simulink model "beaver_agent_env"  (R2022a)
settings: Solver=VariableStepAuto  StartTime=0.0  StopTime=60  FixedStep=1/120  RelTol=1e-5
PreLoadFcn:
  | [aircraft, state] = astDehavillandBeaver();
  | thrustX = getCoefficient(aircraft,"CX","Propeller",Component="Propeller");
  | AileronCmd = 0.00202547955338193;
  | ElevatorCmd = -0.0109658218633661;
  | RudderCmd = -0.0374364069557001;
  | Throttle_Left = 0.16863024396043;
  | Throttle_Right = 0.16863024396043;
model workspace (MATLAB code in the model file + MAT data in the model file):
  inputs0.time = 0
  inputs0.signals(1).dimensions = 1
  inputs0.signals(1).values = -0.104711430294
  inputs0.signals(2).dimensions = 1
  inputs0.signals(2).values = -0.0698725229544
  inputs0.signals(3).dimensions = 1
  inputs0.signals(3).values = -0.000215042330254
  states.time = 0
  states.signals(1).values = 0
  states.signals(1).dimensions = 1
  states.signals(1).label = 'CSTATE'
  states.signals(1).blockName = 'untitled/6DOF EOM/6DOF (Euler Angles)/xe,ye,ze'
  states.signals(1).stateName = 'Xe'
  states.signals(1).inReferencedModel = 0
  states.signals(1).sampleTime = [0 0]
  states.signals(2).values = 0
  states.signals(2).dimensions = 1
  states.signals(2).label = 'CSTATE'
  states.signals(2).blockName = 'untitled/6DOF EOM/6DOF (Euler Angles)/xe,ye,ze'
  states.signals(2).stateName = 'Ye'
  states.signals(2).inReferencedModel = 0
  states.signals(2).sampleTime = [0 0]
  states.signals(3).values = -2202
  states.signals(3).dimensions = 1
  states.signals(3).label = 'CSTATE'
  states.signals(3).blockName = 'untitled/6DOF EOM/6DOF (Euler Angles)/xe,ye,ze'
  states.signals(3).stateName = 'Ze'
  states.signals(3).inReferencedModel = 0
  states.signals(3).sampleTime = [0 0]
  states.signals(4).values = 0.128665353089
  states.signals(4).dimensions = 1
  states.signals(4).label = 'CSTATE'
  states.signals(4).blockName = 'untitled/6DOF EOM/6DOF (Euler Angles)/Calculate DCM &
    | Euler Angles/phi
    | theta
    | psi'
  states.signals(4).stateName = 'phi'
  states.signals(4).inReferencedModel = 0
  states.signals(4).sampleTime = [0 0]
  states.signals(5).values = 0.259337659946
  states.signals(5).dimensions = 1
  states.signals(5).label = 'CSTATE'
  states.signals(5).blockName = 'untitled/6DOF EOM/6DOF (Euler Angles)/Calculate DCM &
    | Euler Angles/phi
    | theta
    | psi'
  states.signals(5).stateName = 'theta'
  states.signals(5).inReferencedModel = 0
  states.signals(5).sampleTime = [0 0]
  states.signals(6).values = -0.178947917154
  states.signals(6).dimensions = 1
  states.signals(6).label = 'CSTATE'
  states.signals(6).blockName = 'untitled/6DOF EOM/6DOF (Euler Angles)/Calculate DCM &
    | Euler Angles/phi
    | theta
    | psi'
  states.signals(6).stateName = 'psi'
  states.signals(6).inReferencedModel = 0
  states.signals(6).sampleTime = [0 0]
  states.signals(7).values = 36.9119692666
  states.signals(7).dimensions = 1
  states.signals(7).label = 'CSTATE'
  states.signals(7).blockName = 'untitled/6DOF EOM/6DOF (Euler Angles)/ub,vb,wb'
  states.signals(7).stateName = 'U'
  states.signals(7).inReferencedModel = 0
  states.signals(7).sampleTime = [0 0]
  states.signals(8).values = 8.10720863264
  states.signals(8).dimensions = 1
  states.signals(8).label = 'CSTATE'
  states.signals(8).blockName = 'untitled/6DOF EOM/6DOF (Euler Angles)/ub,vb,wb'
  states.signals(8).stateName = 'V'
  states.signals(8).inReferencedModel = 0
  states.signals(8).sampleTime = [0 0]
  states.signals(9).values = 8.82591882596
  states.signals(9).dimensions = 1
  states.signals(9).label = 'CSTATE'
  states.signals(9).blockName = 'untitled/6DOF EOM/6DOF (Euler Angles)/ub,vb,wb'
  states.signals(9).stateName = 'W'
  states.signals(9).inReferencedModel = 0
  states.signals(9).sampleTime = [0 0]
  states.signals(10).values = 0
  states.signals(10).dimensions = 1
  states.signals(10).label = 'CSTATE'
  states.signals(10).blockName = 'untitled/6DOF EOM/6DOF (Euler Angles)/p,q,r '
  states.signals(10).stateName = 'p'
  states.signals(10).inReferencedModel = 0
  states.signals(10).sampleTime = [0 0]
  states.signals(11).values = 0
  states.signals(11).dimensions = 1
  states.signals(11).label = 'CSTATE'
  states.signals(11).blockName = 'untitled/6DOF EOM/6DOF (Euler Angles)/p,q,r '
  states.signals(11).stateName = 'q'
  states.signals(11).inReferencedModel = 0
  states.signals(11).sampleTime = [0 0]
  states.signals(12).values = 0
  states.signals(12).dimensions = 1
  states.signals(12).label = 'CSTATE'
  states.signals(12).blockName = 'untitled/6DOF EOM/6DOF (Euler Angles)/p,q,r '
  states.signals(12).stateName = 'r'
  states.signals(12).inReferencedModel = 0
  states.signals(12).sampleTime = [0 0]
  states.signals(13).values = 0
  states.signals(13).dimensions = 1
  states.signals(13).label = 'CSTATE'
  states.signals(13).blockName = 'untitled/PID Controller/Integrator/Continuous/Integrator'
  states.signals(13).stateName = ''
  states.signals(13).inReferencedModel = 0
  states.signals(13).sampleTime = [0 0]
  states.signals(14).values = 0
  states.signals(14).dimensions = 1
  states.signals(14).label = 'CSTATE'
  states.signals(14).blockName = 'untitled/PID Controller/Filter/Cont. Filter/Filter'
  states.signals(14).stateName = ''
  states.signals(14).inReferencedModel = 0
  states.signals(14).sampleTime = [0 0]
  states.signals(15).values = 0
  states.signals(15).dimensions = 1
  states.signals(15).label = 'CSTATE'
  states.signals(15).blockName = 'untitled/PID Controller1/Integrator/Continuous/Integrator'
  states.signals(15).stateName = ''
  states.signals(15).inReferencedModel = 0
  states.signals(15).sampleTime = [0 0]
  states.signals(16).values = 0
  states.signals(16).dimensions = 1
  states.signals(16).label = 'CSTATE'
  states.signals(16).blockName = 'untitled/PID Controller1/Filter/Cont. Filter/Filter'
  states.signals(16).stateName = ''
  states.signals(16).inReferencedModel = 0
  states.signals(16).sampleTime = [0 0]
  states.signals(17).values = [0 0]
  states.signals(17).dimensions = 2
  states.signals(17).label = 'CSTATE'
  states.signals(17).blockName = 'untitled/Environment Model/Dryden Wind Turbulence Model 
    | (Continuous (+q +r))/Filters on velocities/Hwgw(s)/wg_p1'
  states.signals(17).stateName = ''
  states.signals(17).inReferencedModel = 0
  states.signals(17).sampleTime = [0 0]
  states.signals(18).values = [0 0]
  states.signals(18).dimensions = 2
  states.signals(18).label = 'CSTATE'
  states.signals(18).blockName = 'untitled/Environment Model/Dryden Wind Turbulence Model 
    | (Continuous (+q +r))/Filters on velocities/Hwgw(s)/wg_p2'
  states.signals(18).stateName = ''
  states.signals(18).inReferencedModel = 0
  states.signals(18).sampleTime = [0 0]
  states.signals(19).values = [0 0]
  states.signals(19).dimensions = 2
  states.signals(19).label = 'CSTATE'
  states.signals(19).blockName = 'untitled/Environment Model/Dryden Wind Turbulence Model 
    | (Continuous (+q +r))/Filters on velocities/Hvgw(s)/vg_p1'
  states.signals(19).stateName = ''
  states.signals(19).inReferencedModel = 0
  states.signals(19).sampleTime = [0 0]
  states.signals(20).values = [0 0]
  states.signals(20).dimensions = 2
  states.signals(20).label = 'CSTATE'
  states.signals(20).blockName = 'untitled/Environment Model/Dryden Wind Turbulence Model 
    | (Continuous (+q +r))/Filters on velocities/Hvgw(s)/vgw_p2'
  states.signals(20).stateName = ''
  states.signals(20).inReferencedModel = 0
  states.signals(20).sampleTime = [0 0]
  states.signals(21).values = [0 0]
  states.signals(21).dimensions = 2
  states.signals(21).label = 'CSTATE'
  states.signals(21).blockName = 'untitled/Environment Model/Dryden Wind Turbulence Model 
    | (Continuous (+q +r))/Filters on velocities/Hugw(s)/ug_p'
  states.signals(21).stateName = ''
  states.signals(21).inReferencedModel = 0
  states.signals(21).sampleTime = [0 0]
  states.signals(22).values = [0 0]
  states.signals(22).dimensions = 2
  states.signals(22).label = 'CSTATE'
  states.signals(22).blockName = 'untitled/Environment Model/Dryden Wind Turbulence Model 
    | (Continuous (+q +r))/Filters on angular rates/Hrgw/rgw_p'
  states.signals(22).stateName = ''
  states.signals(22).inReferencedModel = 0
  states.signals(22).sampleTime = [0 0]
  states.signals(23).values = [0 0]
  states.signals(23).dimensions = 2
  states.signals(23).label = 'CSTATE'
  states.signals(23).blockName = 'untitled/Environment Model/Dryden Wind Turbulence Model 
    | (Continuous (+q +r))/Filters on angular rates/Hqgw/qgw_p'
  states.signals(23).stateName = ''
  states.signals(23).inReferencedModel = 0
  states.signals(23).sampleTime = [0 0]
  states.signals(24).values = [0 0]
  states.signals(24).dimensions = 2
  states.signals(24).label = 'CSTATE'
  states.signals(24).blockName = 'untitled/Environment Model/Dryden Wind Turbulence Model 
    | (Continuous (+q +r))/Filters on angular rates/Hpgw/pgw_p'
  states.signals(24).stateName = ''
  states.signals(24).inReferencedModel = 0
  states.signals(24).sampleTime = [0 0]
  states0.time = 0
  states0.signals(1).values = [0 0 -2202]
  states0.signals(1).dimensions = 3
  states0.signals(1).label = 'CSTATE'
  states0.signals(1).blockName = 'asb6DOFAirframeTemplate/6DOF EOM/6DOF (Euler Angles)/xe,ye,ze'
  states0.signals(1).stateName = ''
  states0.signals(1).inReferencedModel = 0
  states0.signals(1).sampleTime = [0 0]
  states0.signals(2).values = [0.128665353089 0.259337659946 -0.178947917154]
  states0.signals(2).dimensions = 3
  states0.signals(2).label = 'CSTATE'
  states0.signals(2).blockName = 'asb6DOFAirframeTemplate/6DOF EOM/6DOF (Euler Angles)/Calculate DCM &
    | Euler Angles/phi
    | theta
    | psi'
  states0.signals(2).stateName = ''
  states0.signals(2).inReferencedModel = 0
  states0.signals(2).sampleTime = [0 0]
  states0.signals(3).values = [36.9119692666 8.10720863264 8.82591882596]
  states0.signals(3).dimensions = 3
  states0.signals(3).label = 'CSTATE'
  states0.signals(3).blockName = 'asb6DOFAirframeTemplate/6DOF EOM/6DOF (Euler Angles)/ub,vb,wb'
  states0.signals(3).stateName = ''
  states0.signals(3).inReferencedModel = 0
  states0.signals(3).sampleTime = [0 0]
  states0.signals(4).values = [0 0 0]
  states0.signals(4).dimensions = 3
  states0.signals(4).label = 'CSTATE'
  states0.signals(4).blockName = 'asb6DOFAirframeTemplate/6DOF EOM/6DOF (Euler Angles)/p,q,r '
  states0.signals(4).stateName = ''
  states0.signals(4).inReferencedModel = 0
  states0.signals(4).sampleTime = [0 0]
  states0.signals(5).values = [0 0]
  states0.signals(5).dimensions = 2
  states0.signals(5).label = 'CSTATE'
  states0.signals(5).blockName = 'asb6DOFAirframeTemplate/Environment Model/Dryden Wind Turbulence Model 
    | (Continuous (+q +r))/Filters on velocities/Hwgw(s)/wg_p1'
  states0.signals(5).stateName = ''
  states0.signals(5).inReferencedModel = 0
  states0.signals(5).sampleTime = [0 0]
  states0.signals(6).values = [0 0]
  states0.signals(6).dimensions = 2
  states0.signals(6).label = 'CSTATE'
  states0.signals(6).blockName = 'asb6DOFAirframeTemplate/Environment Model/Dryden Wind Turbulence Model 
    | (Continuous (+q +r))/Filters on velocities/Hwgw(s)/wg_p2'
  states0.signals(6).stateName = ''
  states0.signals(6).inReferencedModel = 0
  states0.signals(6).sampleTime = [0 0]
  states0.signals(7).values = [0 0]
  states0.signals(7).dimensions = 2
  states0.signals(7).label = 'CSTATE'
  states0.signals(7).blockName = 'asb6DOFAirframeTemplate/Environment Model/Dryden Wind Turbulence Model 
    | (Continuous (+q +r))/Filters on velocities/Hvgw(s)/vg_p1'
  states0.signals(7).stateName = ''
  states0.signals(7).inReferencedModel = 0
  states0.signals(7).sampleTime = [0 0]
  states0.signals(8).values = [0 0]
  states0.signals(8).dimensions = 2
  states0.signals(8).label = 'CSTATE'
  states0.signals(8).blockName = 'asb6DOFAirframeTemplate/Environment Model/Dryden Wind Turbulence Model 
    | (Continuous (+q +r))/Filters on velocities/Hvgw(s)/vgw_p2'
  states0.signals(8).stateName = ''
  states0.signals(8).inReferencedModel = 0
  states0.signals(8).sampleTime = [0 0]
  states0.signals(9).values = [0 0]
  states0.signals(9).dimensions = 2
  states0.signals(9).label = 'CSTATE'
  states0.signals(9).blockName = 'asb6DOFAirframeTemplate/Environment Model/Dryden Wind Turbulence Model 
    | (Continuous (+q +r))/Filters on velocities/Hugw(s)/ug_p'
  states0.signals(9).stateName = ''
  states0.signals(9).inReferencedModel = 0
  states0.signals(9).sampleTime = [0 0]
  states0.signals(10).values = [0 0]
  states0.signals(10).dimensions = 2
  states0.signals(10).label = 'CSTATE'
  states0.signals(10).blockName = 'asb6DOFAirframeTemplate/Environment Model/Dryden Wind Turbulence Model 
    | (Continuous (+q +r))/Filters on angular rates/Hrgw/rgw_p'
  states0.signals(10).stateName = ''
  states0.signals(10).inReferencedModel = 0
  states0.signals(10).sampleTime = [0 0]
  states0.signals(11).values = [0 0]
  states0.signals(11).dimensions = 2
  states0.signals(11).label = 'CSTATE'
  states0.signals(11).blockName = 'asb6DOFAirframeTemplate/Environment Model/Dryden Wind Turbulence Model 
    | (Continuous (+q +r))/Filters on angular rates/Hqgw/qgw_p'
  states0.signals(11).stateName = ''
  states0.signals(11).inReferencedModel = 0
  states0.signals(11).sampleTime = [0 0]
  states0.signals(12).values = [0 0]
  states0.signals(12).dimensions = 2
  states0.signals(12).label = 'CSTATE'
  states0.signals(12).blockName = 'asb6DOFAirframeTemplate/Environment Model/Dryden Wind Turbulence Model 
    | (Continuous (+q +r))/Filters on angular rates/Hpgw/pgw_p'
  states0.signals(12).stateName = ''
  states0.signals(12).inReferencedModel = 0
  states0.signals(12).sampleTime = [0 0]
  other statements: initialize6DOFSkyHogg;
values from neighbouring files (symbols this model uses):
  q = double(simOut.q.Data(:))    [apply_twin_trim.m]
  r = double(simOut.r.Data(:))    [apply_twin_trim.m]
  state = read_state(simOut, previousAltitude, stepTime)    [test_300_200_transition.m]
undefined symbols (not defined in the file or in its folder): aircraft, Earth, F, Light, MIL, WGS84
libraries: aerolibasang x4, slpidlib x2, shared6dof x1, aerolibadyn x1, aerolibatmos2 x1, aerolibwind2 x1, aerolibtransform2 x1, sharedtransform x1
settings Model: Creator=Petrichor  LastModifiedBy=velpro
settings SolverCC: AlgebraicLoopSolver=TrustRegion  AutoInsertRateTranBlk=on  InsertRTBMode=Never (minimum delay)  MinimalZcImpactIntegration=on  MaxZcPerStep=1
settings DataIOCC: ExternalInput=inputs0  InitialState=states  SaveFinalState=on  SaveFormat=Array  SaveState=on  LoggingToFile=on
settings OptimizationCC: EnhancedBackFolding=on  StrengthReduction=on  InitFltsAndDblsToZero=on  DifferentSizesBufferReuse=on
settings DebuggingCC: WriteAfterWriteMsg=DisableAll  AlgebraicLoopMsg=none  FcnCallInpInsideContextMsg=warning  UniqueDataStoreMsg=error  RootOutportRequireBusObject=none  StateNameClashWarn=warning  StrictBusMsg=ErrorOnBusTreatedAsVector  SFUnexpectedBacktrackingDiag=warning  SFNoUnconditionalDefaultTransitionDiag=warning  SFExecutionAtInitializationDiag=none  SFMachineParentedDataDiag=warning  ArithmeticOperatorsInVariantConditions=warning
settings ModelReferenceCC: PropagateSignalLabelsOutOfModel=off
settings SFSimCC: SimUseLocalCustomCode=off
settings RTWCC: RTWUseLocalCustomCode=off  DLArmComputeVersion=19.05
settings CodeAppCC: StateflowObjectComments=on

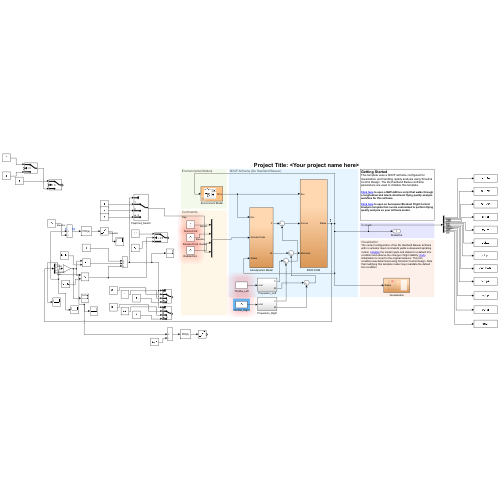
[thumbnail: Simulink's stored preview of the top-level diagram]
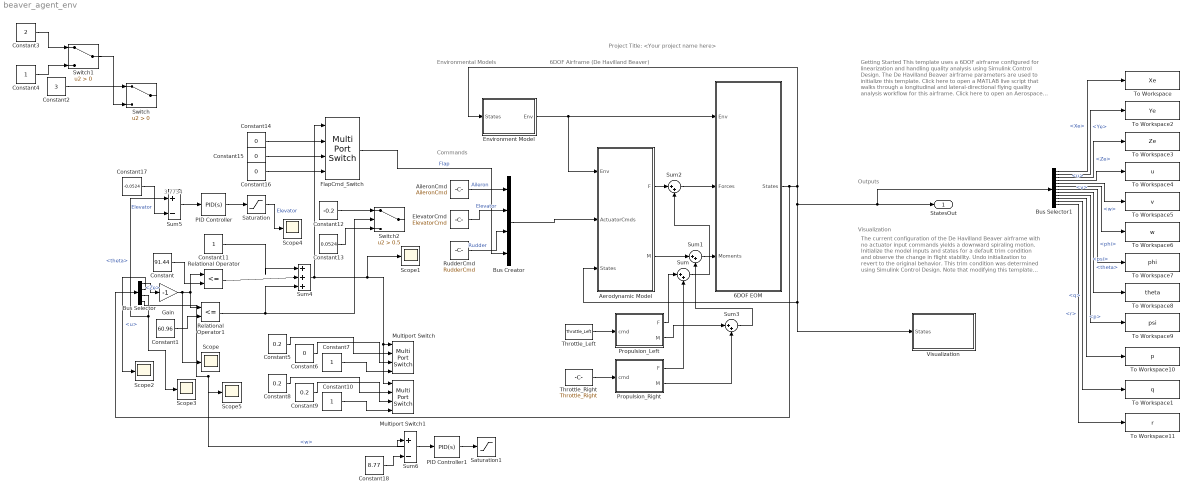
== system beaver_agent_env ==
  note: 3.7734
  note: Project Title: <Your project name here>
  note: 6DOF Airframe (De Havilland Beaver)
  note: Environmental Models
  note: Commands
  note: The current configuration of the De Havilland Beaver airframe with no actuator input commands yields a downward spiraling motion. Initialize the model inputs and states for a default trim condition and observe the change in flight stability. Undo initialization to revert to the original behavior. This trim condition was determined using Simulink Control Design. Note that modifying this template model may invalidate the default trim condition.
  note: Visualization
  note: Outputs
  note: Getting Started
      | This template uses a 6DOF airframe configured for linearization and handling quality analysis using Simulink Control Design. The De Havilland Beaver airframe parameters are used to initialize this template.
      |
      | Click here to open a MATLAB live script that walks through a longitudinal and lateral-directional flying quality analysis workflow for this airframe.
      |
      | Click here to open an Aerospace Blockset Flight Control Analysis template that can be customized to perform flying quality analysis on your airframe model.
  6DOF EOM : Subsystem  VariantControl=eom3DOF
  Aerodynamic Model : Subsystem  VariantControl=aeroCONST
  AileronCmd : Constant  Value=AileronCmd
  Bus Creator : BusCreator  Inputs=4
  Bus Selector : BusSelector  OutputSignals=Ze,u,theta,w
  Bus Selector1 : BusSelector  OutputSignals=Xe,Ye,Ze,u,v,w,phi,theta,psi,p,q,r
  Constant : Constant  Value=91.44
  Constant1 : Constant  Value=60.96
  Constant{4,7,10..11} (4 alike) : Constant
  Constant12 : Constant  Value=-0.2
  Constant13 : Constant  Value=0.0524
  Constant{6,14..16} (4 alike) : Constant  Value=0
  Constant17 : Constant  Value=-0.0524
  Constant18 : Constant  Value=8.77
  Constant2 : Constant  Value=3
  Constant3 : Constant  Value=2
  Constant5 : Constant  Value=0.2
  Constant8 : Constant  Value=0.2
  Constant9 : Constant  Value=0.2
  ElevatorCmd : Constant  Value=ElevatorCmd
  Environment Model : Subsystem  mask(Environment Model){spec=MIL-F-8785C, model=Continuous Dryden (+q -r), W20=5, Wdeg=0, TurbProb=10^-2 - Light, L_high=533.4, Wingspan=4, ts=0.1, Seed=[23341 23342 23343 23344], T_on=off, refAlt=state.GroundHeight}
      mask prompts: spec "aeroblks:aeroblkwind:blockWindTurbulenceModelParamSpecification"; model "aeroblks:aeroblkwind:blockWindTurbulenceModelParamModeltype"; W20 "Wind speed at 6 m defines the low-altitude intensity (m/s):"; Wdeg "Wind direction at 6 m (degrees clockwise from north):"; TurbProb "aeroblks:aeroblkwind:blockWindTurbulenceModelParamProbabilityofexceedanceofhighaltitudeintensity"; L_high "Scale length at medium/high altitudes (m):"; Wingspan "Wingspan (m):"; ts "Band limited noise sample time (sec):"; Seed "aeroblks:aeroblkwind:blockWindTurbulenceModelParamNoiseseedsugvgwgpg"; T_on "aeroblks:aeroblkwind:blockWindTurbulenceModelParamTurbulenceon"; refAlt "Reference height from Earth's surface to Flat Earth frame [m]:"
      mask help: This block contains an athmospheric model, a wind turbulence model, and a gravity model.
      mask Help: helpview(fullfile(docroot,'toolbox','aeroblks','aeroblks.map'), 'environment1');
      mask TypeOptions spec:
      | Dryden Wind Turbulence Model
      | (Continuous (+q +r))/spec
      mask TypeOptions model:
      | Dryden Wind Turbulence Model
      | (Continuous (+q +r))/model
      mask TypeOptions W20:
      | Dryden Wind Turbulence Model
      | (Continuous (+q +r))/W20
      mask TypeOptions Wdeg:
      | Dryden Wind Turbulence Model
      | (Continuous (+q +r))/Wdeg
      mask TypeOptions TurbProb:
      | Dryden Wind Turbulence Model
      | (Continuous (+q +r))/TurbProb
      mask TypeOptions L_high:
      | Dryden Wind Turbulence Model
      | (Continuous (+q +r))/L_high
      mask TypeOptions Wingspan:
      | Dryden Wind Turbulence Model
      | (Continuous (+q +r))/Wingspan
      mask TypeOptions ts:
      | Dryden Wind Turbulence Model
      | (Continuous (+q +r))/ts
      mask TypeOptions Seed:
      | Dryden Wind Turbulence Model
      | (Continuous (+q +r))/Seed
      mask TypeOptions T_on:
      | Dryden Wind Turbulence Model
      | (Continuous (+q +r))/T_on
      mask DialogControl Container4 Prompt: Atmospheric Model
      mask DialogControl Container17 Prompt: 1976 COESA-extended U.S. Standard Atmospheric Model
      mask DialogControl Control6 Prompt: There are no modifiable parameters for COESA.
      mask DialogControl Container6 Prompt: Wind Model
      mask DialogControl Container16 Prompt: Dryden Wind Turbulence Model
      mask DialogControl spec Prompt: Specification:
      mask DialogControl model Prompt: Model type:
      mask DialogControl TurbProb Prompt: Probability of exceedance of high-altitude intensity:
      mask DialogControl Seed Prompt: Noise seeds [ug vg wg pg]:
      mask DialogControl T_on Prompt: Turbulence on
      mask DialogControl Container8 Prompt: Gravity Model
      mask DialogControl Container18 Prompt: World Geodetic System (WGS 84) Gravity Taylor Series Model
      mask Display:
      | image('aeroenvironment.bmp',[.15,.15,.55,.75])
      | port_label('output',1,'Env')
  FlapCmd_Switch : MultiPortSwitch  SaturateOnIntegerOverflow=off  InputSameDT=off
  Gain : Gain  Gain=-1
  Multiport Switch : MultiPortSwitch  SaturateOnIntegerOverflow=off  InputSameDT=off
  Multiport Switch1 : MultiPortSwitch  SaturateOnIntegerOverflow=off  InputSameDT=off
  PID Controller : slpidlib/PID Controller  Controller=PID  Form=Parallel  TimeDomain=Continuous-time  UseExternalTs=off  SampleTime=-1  IntegratorMethod=Forward Euler  FilterMethod=Forward Euler  ControllerParametersSource=internal  P=10  I=2  UseKiTs=off  D=5  N=100  UseFilter=on  TunerSelectOption=Transfer Function Based (PID Tuner App)  InitialConditionSource=internal  InitialConditionForIntegrator=0  InitialConditionForFilter=0  DifferentiatorICPrevScaledInput=0  ExternalReset=none  TrackingMode=off  Kt=1  LimitOutput=off  SatLimitsSource=internal  UpperSaturationLimit=inf  LowerSaturationLimit=-inf  LinearizeAsGain=on  AntiWindupMode=none  Kb=1  POutMin=[]  POutMax=[]  IOutMin=[]  IOutMax=[]  DOutMin=[]  DOutMax=[]  NOutMin=[]  NOutMax=[]  SumOutMin=[]  SumOutMax=[]  SaturationOutMin=[]  SaturationOutMax=[]  PParamMin=[]  PParamMax=[]  IParamMin=[]  IParamMax=[]  DParamMin=[]  DParamMax=[]  NParamMin=[]  NParamMax=[]  KbParamMin=[]  KbParamMax=[]  KtParamMin=[]  KtParamMax=[]  KbOutMin=[]  KbOutMax=[]  KtOutMin=[]  KtOutMax=[]  IntegratorOutMin=[]  IntegratorOutMax=[]  FilterOutMin=[]  FilterOutMax=[]  SumI1OutMin=[]  SumI1OutMax=[]  SumI2OutMin=[]  SumI2OutMax=[]  SumI3OutMin=[]  SumI3OutMax=[]  SumI4OutMin=[]  SumI4OutMax=[]  SumDOutMin=[]  SumDOutMax=[]  DifferentiatorOutMin=[]  DifferentiatorOutMax=[]  FilterDiffOutCoefMin=[]  FilterDiffOutCoefMax=[]  ReciprocalOutMin=[]  ReciprocalOutMax=[]  SumDenOutMin=[]  SumDenOutMax=[]  SumNumOutMin=[]  SumNumOutMax=[]  DivideOutMin=[]  DivideOutMax=[]  UdiffTsProdOutMin=[]  UdiffTsProdOutMax=[]  NTsProdOutMin=[]  NTsProdOutMax=[]  UintegralTsProdOutMin=[]  UintegralTsProdOutMax=[]  UngainTsProdOutMin=[]  UngainTsProdOutMax=[]  IntegratorContinuousStateAttributes=''  IntegratorStateMustResolveToSignalObject=off  IntegratorRTWStateStorageClass=Auto  FilterContinuousStateAttributes=''  FilterStateMustResolveToSignalObject=off  FilterRTWStateStorageClass=Auto  ParallelPVariant=InternalParameters  IdealPVariant=Disabled  IVariant=InternalParameters  DVariant=InternalParameters  IntegratorVariant=Continuous  SatVariant=Disabled  AWVariant=Passthrough  PCopyVariant=Disabled  TRVariant=Disabled  FdbkBlocksVariant=Forward  IdealPFdbkVariant=Disabled  SatFdbkVariant=Disabled  DerivativeFilterVariant=ContFilter  NVariant=InternalParameters  NCopyVariant=Disabled  FilterICVariant=InternalICsFilter  IntegratorICVariant=InternalICs  ExternalResetVariant=Disabled  TRSumVariant=Passthrough  SumFdbkVariant=Disabled  SumVariant=Sum_PID  TsampFilterVariant=InternalTs  TsampNgainVariant=Passthrough  TsampIntegralVariant=Passthrough  ExternalSaturationOutDataTypeStr=Inherit: Same as second input  aMode=0
  PID Controller1 : slpidlib/PID Controller  Controller=PID  Form=Parallel  TimeDomain=Continuous-time  UseExternalTs=off  SampleTime=-1  IntegratorMethod=Forward Euler  FilterMethod=Forward Euler  ControllerParametersSource=internal  P=0.5  I=0.1  UseKiTs=off  D=0.1  N=100  UseFilter=on  TunerSelectOption=Transfer Function Based (PID Tuner App)  InitialConditionSource=internal  InitialConditionForIntegrator=0  InitialConditionForFilter=0  DifferentiatorICPrevScaledInput=0  ExternalReset=none  TrackingMode=off  Kt=1  LimitOutput=off  SatLimitsSource=internal  UpperSaturationLimit=inf  LowerSaturationLimit=-inf  LinearizeAsGain=on  AntiWindupMode=none  Kb=1  POutMin=[]  POutMax=[]  IOutMin=[]  IOutMax=[]  DOutMin=[]  DOutMax=[]  NOutMin=[]  NOutMax=[]  SumOutMin=[]  SumOutMax=[]  SaturationOutMin=[]  SaturationOutMax=[]  PParamMin=[]  PParamMax=[]  IParamMin=[]  IParamMax=[]  DParamMin=[]  DParamMax=[]  NParamMin=[]  NParamMax=[]  KbParamMin=[]  KbParamMax=[]  KtParamMin=[]  KtParamMax=[]  KbOutMin=[]  KbOutMax=[]  KtOutMin=[]  KtOutMax=[]  IntegratorOutMin=[]  IntegratorOutMax=[]  FilterOutMin=[]  FilterOutMax=[]  SumI1OutMin=[]  SumI1OutMax=[]  SumI2OutMin=[]  SumI2OutMax=[]  SumI3OutMin=[]  SumI3OutMax=[]  SumI4OutMin=[]  SumI4OutMax=[]  SumDOutMin=[]  SumDOutMax=[]  DifferentiatorOutMin=[]  DifferentiatorOutMax=[]  FilterDiffOutCoefMin=[]  FilterDiffOutCoefMax=[]  ReciprocalOutMin=[]  ReciprocalOutMax=[]  SumDenOutMin=[]  SumDenOutMax=[]  SumNumOutMin=[]  SumNumOutMax=[]  DivideOutMin=[]  DivideOutMax=[]  UdiffTsProdOutMin=[]  UdiffTsProdOutMax=[]  NTsProdOutMin=[]  NTsProdOutMax=[]  UintegralTsProdOutMin=[]  UintegralTsProdOutMax=[]  UngainTsProdOutMin=[]  UngainTsProdOutMax=[]  IntegratorContinuousStateAttributes=''  IntegratorStateMustResolveToSignalObject=off  IntegratorRTWStateStorageClass=Auto  FilterContinuousStateAttributes=''  FilterStateMustResolveToSignalObject=off  FilterRTWStateStorageClass=Auto  ParallelPVariant=InternalParameters  IdealPVariant=Disabled  IVariant=InternalParameters  DVariant=InternalParameters  IntegratorVariant=Continuous  SatVariant=Disabled  AWVariant=Passthrough  PCopyVariant=Disabled  TRVariant=Disabled  FdbkBlocksVariant=Forward  IdealPFdbkVariant=Disabled  SatFdbkVariant=Disabled  DerivativeFilterVariant=ContFilter  NVariant=InternalParameters  NCopyVariant=Disabled  FilterICVariant=InternalICsFilter  IntegratorICVariant=InternalICs  ExternalResetVariant=Disabled  TRSumVariant=Passthrough  SumFdbkVariant=Disabled  SumVariant=Sum_PID  TsampFilterVariant=InternalTs  TsampNgainVariant=Passthrough  TsampIntegralVariant=Passthrough  ExternalSaturationOutDataTypeStr=Inherit: Same as second input  aMode=0
  Propulsion_Left : Subsystem
      settings: RTWSystemCode=Inline
  Propulsion_Right : Subsystem
      settings: RTWSystemCode=Inline
  Relational Operator : RelationalOperator  Operator=<=  OutDataTypeStr=boolean  RndMeth=Simplest  InputSameDT=off
  Relational Operator1 : RelationalOperator  Operator=<=  OutDataTypeStr=boolean  RndMeth=Simplest  InputSameDT=off
  RudderCmd : Constant  Value=RudderCmd
  Saturation : Saturate  UpperLimit=0.3  LowerLimit=-0.3
  Saturation1 : Saturate  UpperLimit=1  LowerLimit=0
  Scope{,1..5} (6 alike) : Scope
  Sum : Sum  Inputs=|++
  Sum1 : Sum  Inputs=|++  InputSameDT=on  SaturateOnIntegerOverflow=on  OutDataTypeStr=Inherit: Same as first input
  Sum2 : Sum  Inputs=|++  InputSameDT=on  SaturateOnIntegerOverflow=on  OutDataTypeStr=Inherit: Same as first input
  Sum3 : Sum  Inputs=|++
  Sum4 : Sum  Inputs=|+++
  Sum5 : Sum  Inputs=|+-
  Sum6 : Sum  Inputs=|+-
  Switch : Switch  Criteria=u2 > Threshold  SaturateOnIntegerOverflow=off  InputSameDT=off
  Switch1 : Switch  Criteria=u2 > Threshold  SaturateOnIntegerOverflow=off  InputSameDT=off
  Switch2 : Switch  Criteria=u2 > Threshold  Threshold=0.5  SaturateOnIntegerOverflow=off  InputSameDT=off
  Throttle_Left : Constant  Value=Throttle_Left
  Throttle_Right : Constant  Value=Throttle_Right
  To Workspace : ToWorkspace  VariableName=Xe  SaveFormat=Timeseries  SampleTime=-1
  To Workspace1 : ToWorkspace  VariableName=q  SaveFormat=Timeseries  SampleTime=-1
  To Workspace10 : ToWorkspace  VariableName=p  SaveFormat=Timeseries  SampleTime=-1
  To Workspace11 : ToWorkspace  VariableName=r  SaveFormat=Timeseries  SampleTime=-1
  To Workspace2 : ToWorkspace  VariableName=Ye  SaveFormat=Timeseries  SampleTime=-1
  To Workspace3 : ToWorkspace  VariableName=Ze  SaveFormat=Timeseries  SampleTime=-1
  To Workspace4 : ToWorkspace  VariableName=u  SaveFormat=Timeseries  SampleTime=-1
  To Workspace5 : ToWorkspace  VariableName=v  SaveFormat=Timeseries  SampleTime=-1
  To Workspace6 : ToWorkspace  VariableName=w  SaveFormat=Timeseries  SampleTime=-1
  To Workspace7 : ToWorkspace  VariableName=phi  SaveFormat=Timeseries  SampleTime=-1
  To Workspace8 : ToWorkspace  VariableName=theta  SaveFormat=Timeseries  SampleTime=-1
  To Workspace9 : ToWorkspace  VariableName=psi  SaveFormat=Timeseries  SampleTime=-1
  Visualization : Subsystem
  StatesOut : Outport  OutDataTypeStr=double  VectorParamsAs1DForOutWhenUnconnected=off
  wires:
  AileronCmd/1 -> Bus Creator/1  "Aileron"
  RudderCmd/1 -> Bus Creator/3  "Rudder"
  Sum2/1 -> 6DOF EOM/2(Forces)
  Sum1/1 -> 6DOF EOM/3(Moments)
  Aerodynamic Model/1(F) -> Sum2/1
  Aerodynamic Model/2(M) -> Sum1/1
  Environment Model/1(Env) -> 6DOF EOM/1(Env), Aerodynamic Model/1(Env)
  Bus Creator/1 -> Aerodynamic Model/2(ActuatorCmds)
  Propulsion_Left/1(F) -> Sum/1
  Propulsion_Right/1(F) -> Sum/2
  Sum/1 -> Sum2/2
  Propulsion_Left/2(M) -> Sum3/1
  Propulsion_Right/2(M) -> Sum3/2
  Sum3/1 -> Sum1/2
  Bus Selector/1 -> Gain/1  "<Ze>"
  Gain/1 -> Scope/1, Relational Operator1/1, Relational Operator/1
  Constant/1 -> Relational Operator/2
  Constant1/1 -> Relational Operator1/2
  Constant3/1 -> Switch1/1
  Constant4/1 -> Switch1/3
  Constant2/1 -> Switch/1
  Switch1/1 -> Switch/3
  Constant7/1 -> Multiport Switch/4
  Constant6/1 -> Multiport Switch/3
  Constant5/1 -> Multiport Switch/2
  Constant10/1 -> Multiport Switch1/4
  Constant9/1 -> Multiport Switch1/3
  Constant8/1 -> Multiport Switch1/2
  Constant11/1 -> Sum4/1
  Relational Operator/1 -> Sum4/2
  Relational Operator1/1 -> Switch2/2, Sum4/3
  Sum4/1 -> Scope1/1, Multiport Switch1/1, Multiport Switch/1, FlapCmd_Switch/1
  Bus Selector/2 -> Scope2/1  "<u>"
  Constant12/1 -> Switch2/1
  Constant13/1 -> Switch2/3
  Constant16/1 -> FlapCmd_Switch/4
  Constant15/1 -> FlapCmd_Switch/3
  Constant14/1 -> FlapCmd_Switch/2
  FlapCmd_Switch/1 -> Bus Creator/4  "Flap"
  Bus Selector/3 -> Sum5/1, Scope3/1  "<theta>"
  Sum5/1 -> PID Controller/1
  PID Controller/1 -> Saturation/1
  Saturation/1 -> Scope4/1  "Elevator"
  Constant17/1 -> Sum5/2  "Elevator"
  Bus Selector/4 -> Sum6/1, Scope5/1  "<w>"
  Constant18/1 -> Sum6/2
  Sum6/1 -> PID Controller1/1
  PID Controller1/1 -> Saturation1/1
  ElevatorCmd/1 -> Bus Creator/2  "Elevator"
  Throttle_Left/1 -> Propulsion_Left/1(cmd)
  Throttle_Right/1 -> Propulsion_Right/1(cmd)
  Bus Selector1/4 -> To Workspace4/1  "<u>"
  Bus Selector1/6 -> To Workspace6/1  "<w>"
  Bus Selector1/10 -> To Workspace10/1  "<p>"
  Bus Selector1/11 -> To Workspace1/1  "<q>"
  Bus Selector1/7 -> To Workspace7/1  "<phi>"
  Bus Selector1/1 -> To Workspace/1  "<Xe>"
  Bus Selector1/9 -> To Workspace9/1  "<psi>"
  Bus Selector1/2 -> To Workspace2/1  "<Ye>"
  6DOF EOM/1(States) -> Bus Selector/1, Environment Model/1(States), Bus Selector1/1, StatesOut/1, Aerodynamic Model/3(States), Visualization/1(States)
  Bus Selector1/8 -> To Workspace8/1  "<theta>"
  Bus Selector1/12 -> To Workspace11/1  "<r>"
  Bus Selector1/5 -> To Workspace5/1  "<v>"
  Bus Selector1/3 -> To Workspace3/1  "<Ze>"

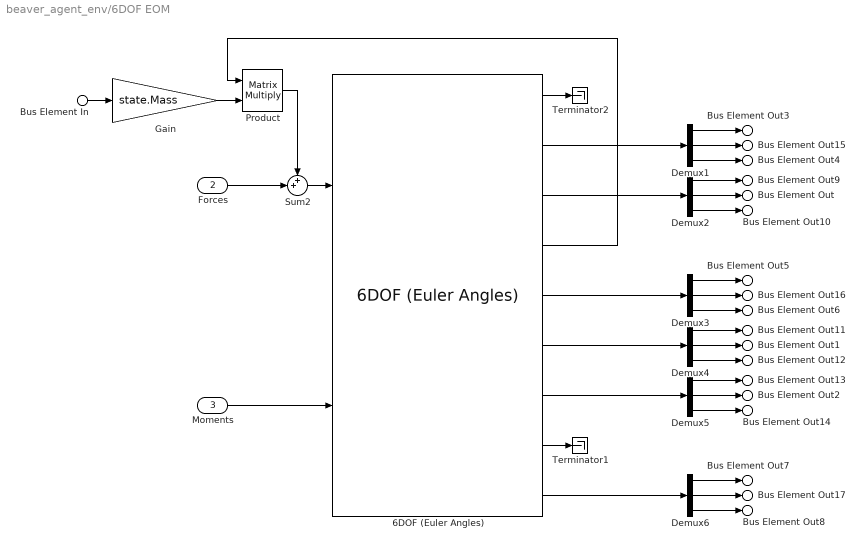
== system beaver_agent_env/6DOF EOM ==
  Bus Element In : Inport  PortName=Env  Element=g
  Forces : Inport  Port=2
  Moments : Inport  Port=3
  6DOF (Euler Angles) : shared6dof/6DOF (Euler Angles)  units=Metric (MKS)  mtype=Fixed  rep=Euler Angles  xme_0=[0 -3.94001921475556e-15 -152.4]  Vm_0=[45 0.0806675282189275 5.92408183813408]  eul_0=[0.0136160413039489 0.0647610681202579 0]  pm_0=[-2.77543447295625e-25 -5.92780243306144e-23 1.72615895877901e-23]  mass_0=state.Mass  mass_e=0.5  mass_f=2.0  inertia=state.Inertia.Variables  inertia_e=eye(3)  inertia_f=2*eye(3)  k_quat=1.0  vre_flag=on  abi_flag=on  aMode=0  xme_statename={'Xe', 'Ye', 'Ze'}  Vm_statename={'U', 'V', 'W'}  eul_statename={'phi', 'theta', 'psi'}  quat_statename={'qr', 'qi', 'qj','qk'}  pm_statename={'p', 'q', 'r'}  mass_statename=''
      settings: SourceProductBaseCode=AE,PW,DR,MT,VE
  Demux{1..6} (6 alike) : Demux  Outputs=3
  Gain : Gain  Gain=state.Mass
  Product : Product  Multiplication=Matrix(*)
  Sum2 : Sum  Inputs=++|  InputSameDT=on  SaturateOnIntegerOverflow=on  OutDataTypeStr=Inherit: Same as first input
  Terminator1 : Terminator
  Terminator2 : Terminator
  Bus Element Out3 : Outport  VectorParamsAs1DForOutWhenUnconnected=off  PortName=States  Element=Xe
  Bus Element Out4 : Outport  VectorParamsAs1DForOutWhenUnconnected=off  PortName=States  Element=Ze
  Bus Element Out : Outport  VectorParamsAs1DForOutWhenUnconnected=off  PortName=States  Element=theta
  Bus Element Out5 : Outport  VectorParamsAs1DForOutWhenUnconnected=off  PortName=States  Element=u
  Bus Element Out6 : Outport  VectorParamsAs1DForOutWhenUnconnected=off  PortName=States  Element=w
  Bus Element Out1 : Outport  VectorParamsAs1DForOutWhenUnconnected=off  PortName=States  Element=q
  Bus Element Out2 : Outport  VectorParamsAs1DForOutWhenUnconnected=off  PortName=States  Element=q_dot
  Bus Element Out7 : Outport  VectorParamsAs1DForOutWhenUnconnected=off  PortName=States  Element=Axe
  Bus Element Out8 : Outport  VectorParamsAs1DForOutWhenUnconnected=off  PortName=States  Element=Aze
  Bus Element Out15 : Outport  VectorParamsAs1DForOutWhenUnconnected=off  PortName=States  Element=Ye
  Bus Element Out9 : Outport  VectorParamsAs1DForOutWhenUnconnected=off  PortName=States  Element=phi
  Bus Element Out10 : Outport  VectorParamsAs1DForOutWhenUnconnected=off  PortName=States  Element=psi
  Bus Element Out16 : Outport  VectorParamsAs1DForOutWhenUnconnected=off  PortName=States  Element=v
  Bus Element Out11 : Outport  VectorParamsAs1DForOutWhenUnconnected=off  PortName=States  Element=p
  Bus Element Out12 : Outport  VectorParamsAs1DForOutWhenUnconnected=off  PortName=States  Element=r
  Bus Element Out13 : Outport  VectorParamsAs1DForOutWhenUnconnected=off  PortName=States  Element=p_dot
  Bus Element Out14 : Outport  VectorParamsAs1DForOutWhenUnconnected=off  PortName=States  Element=r_dot
  Bus Element Out17 : Outport  VectorParamsAs1DForOutWhenUnconnected=off  PortName=States  Element=Aye
  wires:
  6DOF (Euler Angles)/2 -> Demux1/1
  6DOF (Euler Angles)/4 -> Product/1
  6DOF (Euler Angles)/1 -> Terminator2/1
  Bus Element In/1 -> Gain/1
  Demux6/2 -> Bus Element Out17/1
  Demux6/3 -> Bus Element Out8/1
  Demux6/1 -> Bus Element Out7/1
  6DOF (Euler Angles)/9 -> Demux6/1
  6DOF (Euler Angles)/7 -> Demux5/1
  Demux5/3 -> Bus Element Out14/1
  Demux5/2 -> Bus Element Out2/1
  Demux5/1 -> Bus Element Out13/1
  6DOF (Euler Angles)/6 -> Demux4/1
  Demux4/3 -> Bus Element Out12/1
  Demux4/2 -> Bus Element Out1/1
  Demux4/1 -> Bus Element Out11/1
  Demux3/3 -> Bus Element Out6/1
  Demux3/2 -> Bus Element Out16/1
  Demux3/1 -> Bus Element Out5/1
  6DOF (Euler Angles)/5 -> Demux3/1
  Demux2/3 -> Bus Element Out10/1
  Demux2/2 -> Bus Element Out/1
  Demux2/1 -> Bus Element Out9/1
  Demux1/1 -> Bus Element Out3/1
  Demux1/3 -> Bus Element Out4/1
  Demux1/2 -> Bus Element Out15/1
  Gain/1 -> Product/2
  6DOF (Euler Angles)/3 -> Demux2/1
  Moments/1 -> 6DOF (Euler Angles)/2
  Forces/1 -> Sum2/2
  Sum2/1 -> 6DOF (Euler Angles)/1
  Product/1 -> Sum2/1
  6DOF (Euler Angles)/8 -> Terminator1/1

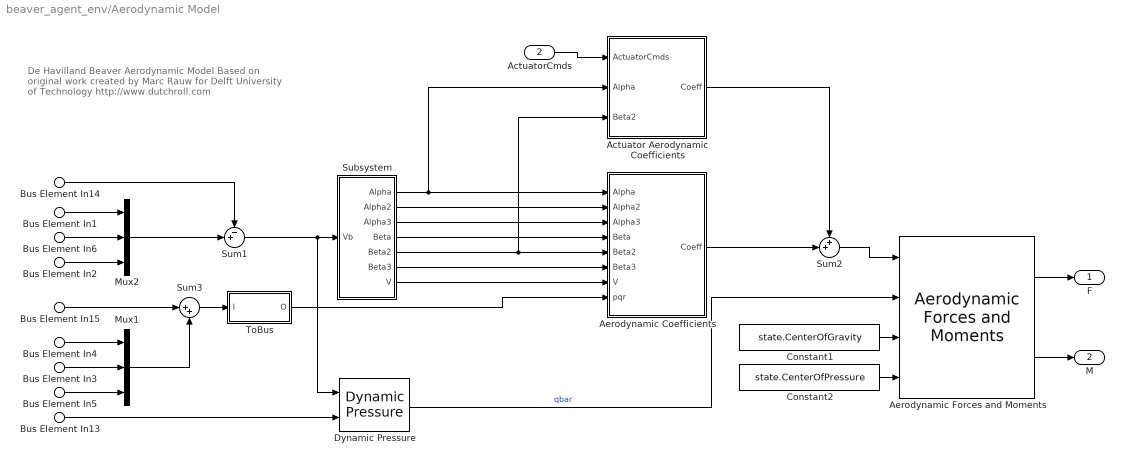
== system beaver_agent_env/Aerodynamic Model ==
  note: De Havilland Beaver Aerodynamic Model
      | Based on original work created by
      | Marc Rauw for Delft University of Technology
      | http://www.dutchroll.com
  Bus Element In13 : Inport  PortName=Env  Element=AirDensity
  Bus Element In14 : Inport  PortName=Env  Element=WindVelocity
  Bus Element In15 : Inport  PortName=Env  Element=WindAngularRates
  ActuatorCmds : Inport  Port=2
  Bus Element In1 : Inport  Port=3  PortName=States  Element=u
  Bus Element In2 : Inport  Port=3  PortName=States  Element=w
  Bus Element In3 : Inport  Port=3  PortName=States  Element=q
  Bus Element In6 : Inport  Port=3  PortName=States  Element=v
  Bus Element In4 : Inport  Port=3  PortName=States  Element=p
  Bus Element In5 : Inport  Port=3  PortName=States  Element=r
  Actuator Aerodynamic Coefficients : Subsystem
  Aerodynamic Coefficients : Subsystem
  Aerodynamic Forces and Moments : aerolibadyn/Aerodynamic Forces and Moments   inputAxes=Body  outputForceAxes=Body  outputMomentAxes=Body  S=aircraft.ReferenceArea  b=aircraft.ReferenceSpan  cbar=aircraft.ReferenceLength
  Constant1 : Constant  Value=state.CenterOfGravity
  Constant2 : Constant  Value=state.CenterOfPressure
  Dynamic Pressure : aerolibasang/Dynamic Pressure
  Mux1 : Mux  Inputs=3
  Mux2 : Mux  Inputs=3
  Subsystem : Subsystem
  Sum1 : Sum  Inputs=-+|  InputSameDT=on  SaturateOnIntegerOverflow=on  OutDataTypeStr=Inherit: Same as first input
  Sum2 : Sum  Inputs=++|
  Sum3 : Sum  Inputs=|++  InputSameDT=on  SaturateOnIntegerOverflow=on  OutDataTypeStr=Inherit: Same as first input
  ToBus : Subsystem
  F : Outport  Unit=N  VectorParamsAs1DForOutWhenUnconnected=off
  M : Outport  Port=2  Unit=N*m  VectorParamsAs1DForOutWhenUnconnected=off
  wires:
  ActuatorCmds/1 -> Actuator Aerodynamic Coefficients/1(ActuatorCmds)
  Bus Element In14/1 -> Sum1/1
  Mux2/1 -> Sum1/2
  Mux1/1 -> Sum3/2
  Bus Element In15/1 -> Sum3/1
  Bus Element In5/1 -> Mux1/3
  Bus Element In3/1 -> Mux1/2
  Bus Element In4/1 -> Mux1/1
  Actuator Aerodynamic Coefficients/1(Coeff) -> Sum2/1
  Aerodynamic Coefficients/1(Coeff) -> Sum2/2
  ToBus/1(O) -> Aerodynamic Coefficients/8(pqr)
  Sum1/1 -> Dynamic Pressure/1, Subsystem/1(Vb)
  Dynamic Pressure/1 -> Aerodynamic Forces and Moments/2  "qbar"
  Sum3/1 -> ToBus/1(I)
  Bus Element In13/1 -> Dynamic Pressure/2
  Subsystem/7(V) -> Aerodynamic Coefficients/7(V)
  Subsystem/4(Beta) -> Aerodynamic Coefficients/4(Beta)
  Aerodynamic Forces and Moments/2 -> M/1
  Aerodynamic Forces and Moments/1 -> F/1
  Constant2/1 -> Aerodynamic Forces and Moments/4
  Constant1/1 -> Aerodynamic Forces and Moments/3
  Sum2/1 -> Aerodynamic Forces and Moments/1
  Bus Element In1/1 -> Mux2/1
  Bus Element In6/1 -> Mux2/2
  Bus Element In2/1 -> Mux2/3
  Subsystem/1(Alpha) -> Aerodynamic Coefficients/1(Alpha), Actuator Aerodynamic Coefficients/2(Alpha)
  Subsystem/5(Beta2) -> Aerodynamic Coefficients/5(Beta2), Actuator Aerodynamic Coefficients/3(Beta2)
  Subsystem/2(Alpha2) -> Aerodynamic Coefficients/2(Alpha2)
  Subsystem/3(Alpha3) -> Aerodynamic Coefficients/3(Alpha3)
  Subsystem/6(Beta3) -> Aerodynamic Coefficients/6(Beta3)

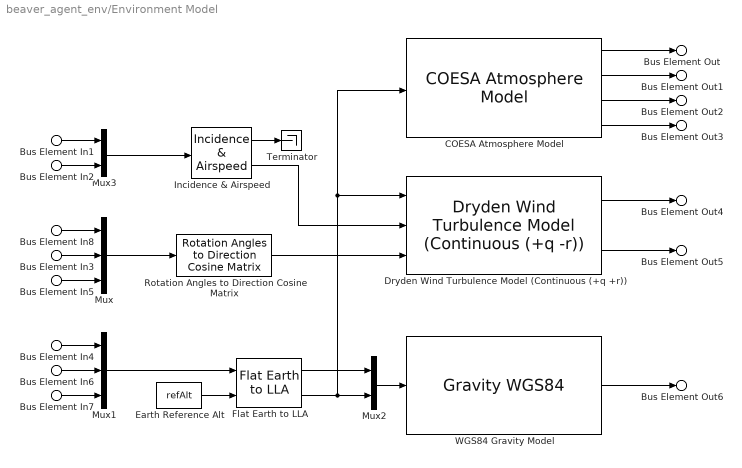
== system beaver_agent_env/Environment Model ==
  Bus Element In1 : Inport  PortName=States  Element=u
  Bus Element In2 : Inport  PortName=States  Element=w
  Bus Element In3 : Inport  PortName=States  Element=theta
  Bus Element In4 : Inport  PortName=States  Element=Xe
  Bus Element In7 : Inport  PortName=States  Element=Ze
  Bus Element In8 : Inport  PortName=States  Element=phi
  Bus Element In5 : Inport  PortName=States  Element=psi
  Bus Element In6 : Inport  PortName=States  Element=Ye
  COESA Atmosphere Model : aerolibatmos2/COESA Atmosphere Model  units=Metric (MKS)  spec=1976 COESA-extended U.S. Standard Atmosphere  model=Profile  profile_var=High temperature  profile_percent=1%  profile_alt=5 km (16404 ft)  envelope_var=High temperature  envelope_percent=1%  action=Warning
  Dryden Wind Turbulence Model (Continuous (+q +r)) : aerolibwind2/Dryden Wind Turbulence Model  (Continuous (+q -r))  units=Metric (MKS)  spec=MIL-F-8785C  model=Continuous Dryden (+q -r)  W20=W20  Wdeg=Wdeg  TurbProb=10^-2 - Light  L_high=L_high  Wingspan=Wingspan  ts=ts  Seed=Seed  T_on=off
  Earth Reference Alt : Constant  Value=refAlt
  Flat Earth to LLA : aerolibtransform2/Flat Earth to LLA  units=Metric (MKS)  ptype=Earth (WGS84)  F=1/298.257223563  R=6378137  refPosPort=off  LL0=[0 0]  psi=0
  Incidence & Airspeed : aerolibasang/Incidence  & Airspeed
      settings: SourceProductBaseCode=AE
  Mux : Mux  Inputs=3
  Mux1 : Mux  Inputs=3
  Mux2 : Mux  Inputs=2
  Mux3 : Mux  Inputs=2
  Rotation Angles to Direction Cosine Matrix : sharedtransform/Rotation Angles to Direction Cosine Matrix  rotationOrder=ZYX  aMode=aMode
      settings: SourceProductBaseCode=AE,PW,DR,MT,VE
  Terminator : Terminator
  "WGS84 Gravity Model  " : GravityWGS84
  Bus Element Out : Outport  VectorParamsAs1DForOutWhenUnconnected=off  PortName=Env  Element=To
  Bus Element Out1 : Outport  VectorParamsAs1DForOutWhenUnconnected=off  PortName=Env  Element=a
  Bus Element Out2 : Outport  VectorParamsAs1DForOutWhenUnconnected=off  PortName=Env  Element=Po
  Bus Element Out3 : Outport  VectorParamsAs1DForOutWhenUnconnected=off  PortName=Env  Element=AirDensity
  Bus Element Out4 : Outport  VectorParamsAs1DForOutWhenUnconnected=off  PortName=Env  Element=WindVelocity
  Bus Element Out5 : Outport  VectorParamsAs1DForOutWhenUnconnected=off  PortName=Env  Element=WindAngularRates
  Bus Element Out6 : Outport  VectorParamsAs1DForOutWhenUnconnected=off  PortName=Env  Element=g
  wires:
  Dryden Wind Turbulence Model (Continuous (+q +r))/1 -> Bus Element Out4/1
  Dryden Wind Turbulence Model (Continuous (+q +r))/2 -> Bus Element Out5/1
  Mux2/1 -> "WGS84 Gravity Model  "/1
  Bus Element In4/1 -> Mux1/1
  Bus Element In7/1 -> Mux1/3
  Bus Element In6/1 -> Mux1/2
  Bus Element In5/1 -> Mux/3
  Bus Element In8/1 -> Mux/1
  Bus Element In2/1 -> Mux3/2
  Bus Element In1/1 -> Mux3/1
  "WGS84 Gravity Model  "/1 -> Bus Element Out6/1
  COESA Atmosphere Model/2 -> Bus Element Out1/1
  COESA Atmosphere Model/1 -> Bus Element Out/1
  COESA Atmosphere Model/4 -> Bus Element Out3/1
  COESA Atmosphere Model/3 -> Bus Element Out2/1
  Flat Earth to LLA/1 -> Mux2/1
  Earth Reference Alt/1 -> Flat Earth to LLA/2
  Incidence & Airspeed/2 -> Dryden Wind Turbulence Model (Continuous (+q +r))/2
  Flat Earth to LLA/2 -> Mux2/2, COESA Atmosphere Model/1, Dryden Wind Turbulence Model (Continuous (+q +r))/1
  Mux3/1 -> Incidence & Airspeed/1
  Incidence & Airspeed/1 -> Terminator/1
  Mux/1 -> Rotation Angles to Direction Cosine Matrix/1
  Bus Element In3/1 -> Mux/2
  Rotation Angles to Direction Cosine Matrix/1 -> Dryden Wind Turbulence Model (Continuous (+q +r))/3
  Mux1/1 -> Flat Earth to LLA/1

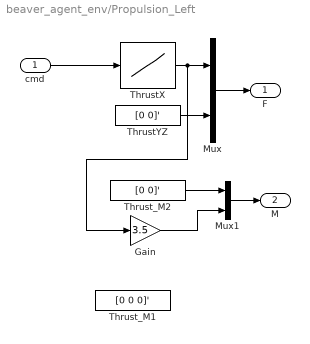
== system beaver_agent_env/Propulsion_Left ==
  cmd : Inport
  Gain : Gain  Gain=3.5
  Mux : Mux  Inputs=[1 2]
  Mux1 : Mux  Inputs=2
  ThrustX : Lookup_n-D  NumberOfTableDimensions=1  LookupTableObject=thrustX  BreakpointsForDimension1="getCoefficient(aircraft,\"CX\",\"Propeller\",Component=\"Propeller\").Breakpoints(1).Value"  IndexSearchMethod=Linear search  BeginIndexSearchUsingPreviousIndexResult=on  Table="[0, 0.75*getCoefficient(aircraft,\"CX\",\"Propeller\",Component=\"Propeller\").Table.Value(2:end)]"  ExtrapMethod=Clip
  ThrustYZ : Constant  Value=[0 0]'  SampleTime=-1
  Thrust_M1 : Constant  Value=[0 0 0]'  SampleTime=-1
  Thrust_M2 : Constant  Value=[0 0]'  SampleTime=-1
  F : Outport  Unit=N  VectorParamsAs1DForOutWhenUnconnected=off
  M : Outport  Port=2  Unit=N*m  VectorParamsAs1DForOutWhenUnconnected=off
  wires:
  ThrustX/1 -> Gain/1, Mux/1
  ThrustYZ/1 -> Mux/2
  Mux/1 -> F/1
  cmd/1 -> ThrustX/1
  Mux1/1 -> M/1
  Thrust_M2/1 -> Mux1/1
  Gain/1 -> Mux1/2

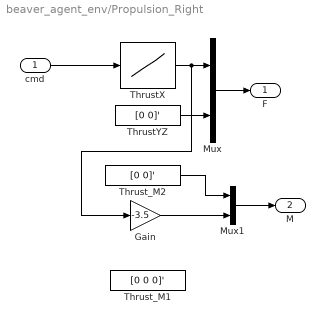
== system beaver_agent_env/Propulsion_Right ==
  cmd : Inport
  Gain : Gain  Gain=-3.5
  Mux : Mux  Inputs=[1 2]
  Mux1 : Mux  Inputs=2
  ThrustX : Lookup_n-D  NumberOfTableDimensions=1  LookupTableObject=thrustX  BreakpointsForDimension1="getCoefficient(aircraft,\"CX\",\"Propeller\",Component=\"Propeller\").Breakpoints(1).Value"  IndexSearchMethod=Linear search  BeginIndexSearchUsingPreviousIndexResult=on  Table="[0, 0.75*getCoefficient(aircraft,\"CX\",\"Propeller\",Component=\"Propeller\").Table.Value(2:end)]"  ExtrapMethod=Clip
  ThrustYZ : Constant  Value=[0 0]'  SampleTime=-1
  Thrust_M1 : Constant  Value=[0 0 0]'  SampleTime=-1
  Thrust_M2 : Constant  Value=[0 0]'  SampleTime=-1
  F : Outport  Unit=N  VectorParamsAs1DForOutWhenUnconnected=off
  M : Outport  Port=2  Unit=N*m  VectorParamsAs1DForOutWhenUnconnected=off
  wires:
  ThrustX/1 -> Gain/1, Mux/1
  ThrustYZ/1 -> Mux/2
  Mux/1 -> F/1
  cmd/1 -> ThrustX/1
  Mux1/1 -> M/1
  Thrust_M2/1 -> Mux1/1
  Gain/1 -> Mux1/2

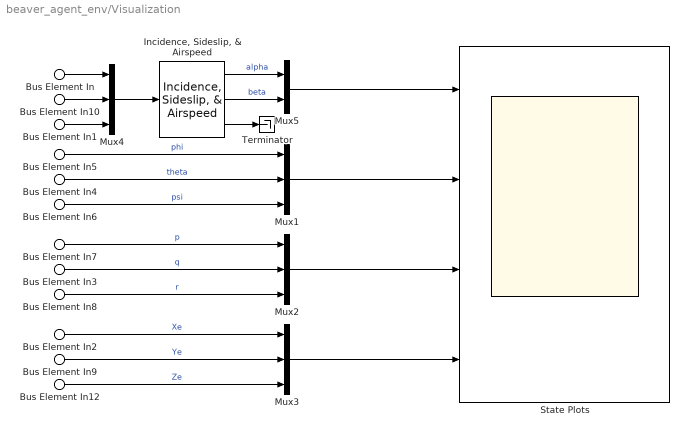
== system beaver_agent_env/Visualization ==
  Bus Element In : Inport  PortName=States  Element=u
  Bus Element In1 : Inport  PortName=States  Element=w
  Bus Element In3 : Inport  PortName=States  Element=q
  Bus Element In4 : Inport  PortName=States  Element=theta
  Bus Element In12 : Inport  PortName=States  Element=Ze
  Bus Element In2 : Inport  PortName=States  Element=Xe
  Bus Element In10 : Inport  PortName=States  Element=v
  Bus Element In5 : Inport  PortName=States  Element=phi
  Bus Element In6 : Inport  PortName=States  Element=psi
  Bus Element In7 : Inport  PortName=States  Element=p
  Bus Element In8 : Inport  PortName=States  Element=r
  Bus Element In9 : Inport  PortName=States  Element=Ye
  "Incidence, Sideslip, & Airspeed" : aerolibasang/Incidence, Sideslip, & Airspeed
  Mux{1..4} (4 alike) : Mux  Inputs=3
  Mux5 : Mux  Inputs=2
  State Plots : Scope  NumInputPorts=4
  Terminator : Terminator
  wires:
  Mux3/1 -> State Plots/4
  Bus Element In2/1 -> Mux3/1  "Xe"
  Bus Element In9/1 -> Mux3/2  "Ye"
  Bus Element In12/1 -> Mux3/3  "Ze"
  Mux2/1 -> State Plots/3
  Mux1/1 -> State Plots/2
  Mux5/1 -> State Plots/1
  "Incidence, Sideslip, & Airspeed"/2 -> Mux5/2  "beta"
  "Incidence, Sideslip, & Airspeed"/1 -> Mux5/1  "alpha"
  Mux4/1 -> "Incidence, Sideslip, & Airspeed"/1
  Bus Element In10/1 -> Mux4/2
  Bus Element In8/1 -> Mux2/3  "r"
  Bus Element In7/1 -> Mux2/1  "p"
  Bus Element In6/1 -> Mux1/3  "psi"
  Bus Element In5/1 -> Mux1/1  "phi"
  Bus Element In4/1 -> Mux1/2  "theta"
  Bus Element In3/1 -> Mux2/2  "q"
  Bus Element In1/1 -> Mux4/3
  Bus Element In/1 -> Mux4/1
  "Incidence, Sideslip, & Airspeed"/3 -> Terminator/1

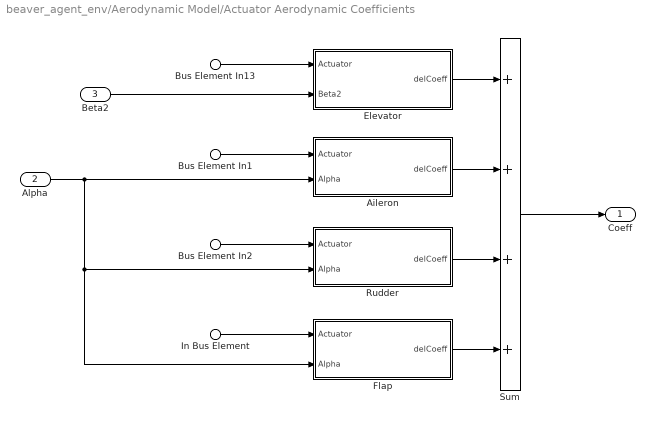
== system beaver_agent_env/Aerodynamic Model/Actuator Aerodynamic Coefficients ==
  Bus Element In13 : Inport  PortName=ActuatorCmds  Element=Elevator
  Bus Element In1 : Inport  PortName=ActuatorCmds  Element=Aileron
  Bus Element In2 : Inport  PortName=ActuatorCmds  Element=Rudder
  In Bus Element : Inport  PortName=ActuatorCmds  Element=Flap
  Alpha : Inport  Port=2
  Beta2 : Inport  Port=3
  Aileron : Subsystem
  Elevator : Subsystem
  Flap : Subsystem
  Rudder : Subsystem
  Sum : Sum  Inputs=4  InputSameDT=on  SaturateOnIntegerOverflow=on  OutDataTypeStr=Inherit: Same as first input
  Coeff : Outport  InitialOutput=0  VectorParamsAs1DForOutWhenUnconnected=off
  wires:
  Bus Element In2/1 -> Rudder/1(Actuator)
  Bus Element In1/1 -> Aileron/1(Actuator)
  Bus Element In13/1 -> Elevator/1(Actuator)
  Beta2/1 -> Elevator/2(Beta2)
  Flap/1(delCoeff) -> Sum/4
  Alpha/1 -> Flap/2(Alpha), Rudder/2(Alpha), Aileron/2(Alpha)
  Rudder/1(delCoeff) -> Sum/3
  Aileron/1(delCoeff) -> Sum/2
  Elevator/1(delCoeff) -> Sum/1
  Sum/1 -> Coeff/1
  In Bus Element/1 -> Flap/1(Actuator)

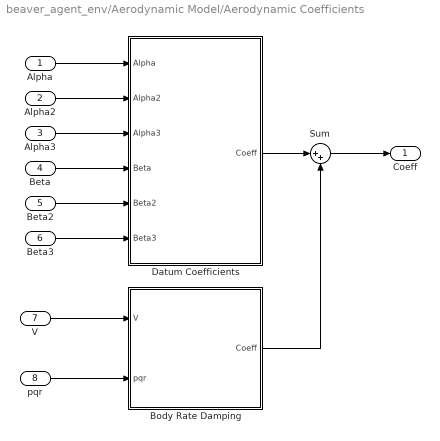
== system beaver_agent_env/Aerodynamic Model/Aerodynamic Coefficients ==
  Alpha : Inport
  Alpha2 : Inport  Port=2
  Alpha3 : Inport  Port=3
  Beta : Inport  Port=4
  Beta2 : Inport  Port=5
  Beta3 : Inport  Port=6
  V : Inport  Port=7
  pqr : Inport  Port=8  Unit=m/s
  Body Rate Damping : Subsystem
  Datum Coefficients : Subsystem
  Sum : Sum  Inputs=|++
  Coeff : Outport  VectorParamsAs1DForOutWhenUnconnected=off
  wires:
  pqr/1 -> Body Rate Damping/2(pqr)
  Sum/1 -> Coeff/1
  V/1 -> Body Rate Damping/1(V)
  Body Rate Damping/1(Coeff) -> Sum/2
  Datum Coefficients/1(Coeff) -> Sum/1
  Beta/1 -> Datum Coefficients/4(Beta)
  Alpha/1 -> Datum Coefficients/1(Alpha)
  Alpha2/1 -> Datum Coefficients/2(Alpha2)
  Alpha3/1 -> Datum Coefficients/3(Alpha3)
  Beta2/1 -> Datum Coefficients/5(Beta2)
  Beta3/1 -> Datum Coefficients/6(Beta3)

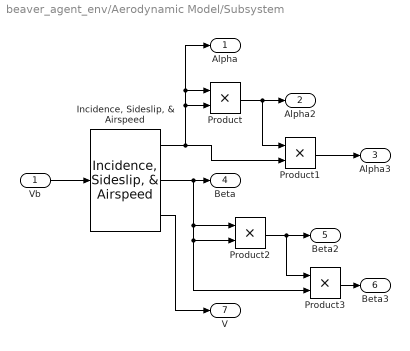
== system beaver_agent_env/Aerodynamic Model/Subsystem ==
  Vb : Inport
  "Incidence, Sideslip, & Airspeed" : aerolibasang/Incidence, Sideslip, & Airspeed
  Product{,1..3} (4 alike) : Product
  Alpha : Outport
  Alpha2 : Outport  Port=2
  Alpha3 : Outport  Port=3
  Beta : Outport  Port=4
  Beta2 : Outport  Port=5
  Beta3 : Outport  Port=6
  V : Outport  Port=7
  wires:
  Product/1 -> Product1/1, Alpha2/1
  "Incidence, Sideslip, & Airspeed"/1 -> Product/1, Alpha/1, Product/2, Product1/2
  "Incidence, Sideslip, & Airspeed"/3 -> V/1
  Vb/1 -> "Incidence, Sideslip, & Airspeed"/1
  Product1/1 -> Alpha3/1
  Product2/1 -> Product3/1, Beta2/1
  Product3/1 -> Beta3/1
  "Incidence, Sideslip, & Airspeed"/2 -> Product3/2, Product2/2, Product2/1, Beta/1

== system beaver_agent_env/Aerodynamic Model/ToBus ==
  I : Inport
  Bus Creator3 : BusCreator  Inputs=3
  Demux : Demux  Outputs=3
  O : Outport  VectorParamsAs1DForOutWhenUnconnected=off
  wires:
  I/1 -> Demux/1
  Demux/2 -> Bus Creator3/2  "q_wind"
  Bus Creator3/1 -> O/1
  Demux/3 -> Bus Creator3/3  "r_wind"
  Demux/1 -> Bus Creator3/1  "p_wind"

== system beaver_agent_env/Aerodynamic Model/Actuator Aerodynamic Coefficients/Aileron ==
  Actuator : Inport
  Alpha : Inport  Port=2
  Constant : Constant  Value=aircraft.Surfaces(1).Surfaces(1).Coefficients.Table.Variables
  Matrix Multiply : Product  Multiplication=Matrix(*)
  Product : Product
  Vector Concatenate : Concatenate
  delCoeff : Outport  VectorParamsAs1DForOutWhenUnconnected=off
  wires:
  Actuator/1 -> Product/1, Vector Concatenate/1
  Alpha/1 -> Product/2
  Vector Concatenate/1 -> Matrix Multiply/2
  Matrix Multiply/1 -> delCoeff/1
  Product/1 -> Vector Concatenate/2
  Constant/1 -> Matrix Multiply/1

== system beaver_agent_env/Aerodynamic Model/Actuator Aerodynamic Coefficients/Elevator ==
  Actuator : Inport
  Beta2 : Inport  Port=2
  Constant : Constant  Value=aircraft.Surfaces(2).Surfaces(1).Coefficients.Table.Variables
  Matrix Multiply : Product  Multiplication=Matrix(*)
  Product : Product
  Vector Concatenate : Concatenate
  delCoeff : Outport  VectorParamsAs1DForOutWhenUnconnected=off
  wires:
  Matrix Multiply/1 -> delCoeff/1
  Constant/1 -> Matrix Multiply/1
  Vector Concatenate/1 -> Matrix Multiply/2
  Actuator/1 -> Product/1, Vector Concatenate/1
  Beta2/1 -> Product/2
  Product/1 -> Vector Concatenate/2

== system beaver_agent_env/Aerodynamic Model/Actuator Aerodynamic Coefficients/Flap ==
  Actuator : Inport
  Alpha : Inport  Port=2
  Constant : Constant  Value=aircraft.Surfaces(1).Surfaces(2).Coefficients.Table.Variables
  Matrix Multiply : Product  Multiplication=Matrix(*)
  Product : Product
  Vector Concatenate : Concatenate
  delCoeff : Outport  VectorParamsAs1DForOutWhenUnconnected=off
  wires:
  Actuator/1 -> Product/1, Vector Concatenate/1
  Alpha/1 -> Product/2
  Vector Concatenate/1 -> Matrix Multiply/2
  Matrix Multiply/1 -> delCoeff/1
  Product/1 -> Vector Concatenate/2
  Constant/1 -> Matrix Multiply/1

== system beaver_agent_env/Aerodynamic Model/Actuator Aerodynamic Coefficients/Rudder ==
  Actuator : Inport
  Alpha : Inport  Port=2
  Constant : Constant  Value=aircraft.Surfaces(3).Surfaces(1).Coefficients.Table.Variables
  Matrix Multiply : Product  Multiplication=Matrix(*)
  Product : Product
  Vector Concatenate : Concatenate
  delCoeff : Outport  VectorParamsAs1DForOutWhenUnconnected=off
  wires:
  Actuator/1 -> Product/1, Vector Concatenate/1
  Alpha/1 -> Product/2
  Vector Concatenate/1 -> Matrix Multiply/2
  Matrix Multiply/1 -> delCoeff/1
  Product/1 -> Vector Concatenate/2
  Constant/1 -> Matrix Multiply/1

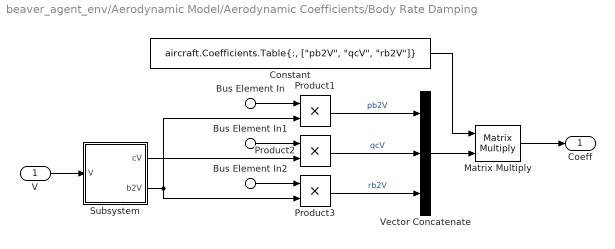
== system beaver_agent_env/Aerodynamic Model/Aerodynamic Coefficients/Body Rate Damping ==
  V : Inport  Unit=m/s
  Bus Element In : Inport  Port=2  PortName=pqr  Element=p_wind
  Bus Element In1 : Inport  Port=2  PortName=pqr  Element=q_wind
  Bus Element In2 : Inport  Port=2  PortName=pqr  Element=r_wind
  Constant : Constant  Value="aircraft.Coefficients.Table{:, [\"pb2V\", \"qcV\", \"rb2V\"]}"
  Matrix Multiply : Product  Multiplication=Matrix(*)
  Product1 : Product
  Product2 : Product
  Product3 : Product
  Subsystem : Subsystem
  Vector Concatenate : Concatenate  NumInputs=3
  Coeff : Outport  InitialOutput=0  VectorParamsAs1DForOutWhenUnconnected=off
  wires:
  Matrix Multiply/1 -> Coeff/1
  Vector Concatenate/1 -> Matrix Multiply/2
  Product1/1 -> Vector Concatenate/1  "pb2V"
  Bus Element In/1 -> Product1/1
  Product2/1 -> Vector Concatenate/2  "qcV"
  Subsystem/2(b2V) -> Product3/2, Product1/2
  Product3/1 -> Vector Concatenate/3  "rb2V"
  Constant/1 -> Matrix Multiply/1
  Bus Element In1/1 -> Product2/1
  Subsystem/1(cV) -> Product2/2
  Bus Element In2/1 -> Product3/1
  V/1 -> Subsystem/1(V)

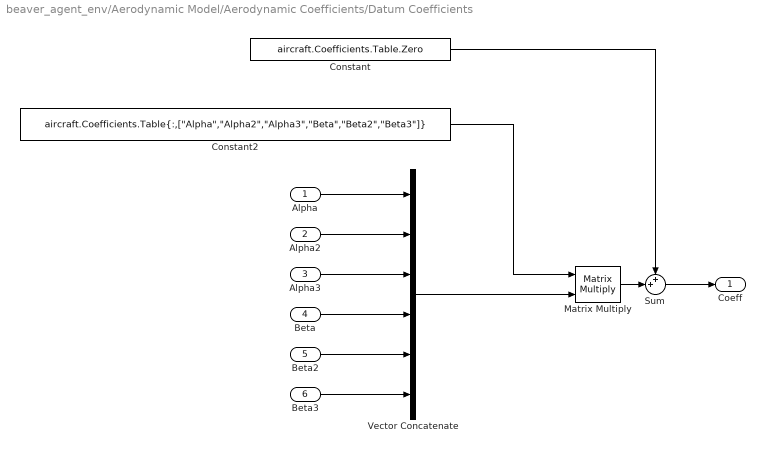
== system beaver_agent_env/Aerodynamic Model/Aerodynamic Coefficients/Datum Coefficients ==
  Alpha : Inport
  Alpha2 : Inport  Port=2
  Alpha3 : Inport  Port=3
  Beta : Inport  Port=4
  Beta2 : Inport  Port=5
  Beta3 : Inport  Port=6
  Constant : Constant  Value=aircraft.Coefficients.Table.Zero
  Constant2 : Constant  Value="aircraft.Coefficients.Table{:,[\"Alpha\",\"Alpha2\",\"Alpha3\",\"Beta\",\"Beta2\",\"Beta3\"]}"
  Matrix Multiply : Product  Multiplication=Matrix(*)
  Sum : Sum  Inputs=++|
  Vector Concatenate : Concatenate  NumInputs=6
  Coeff : Outport  InitialOutput=0  VectorParamsAs1DForOutWhenUnconnected=off
  wires:
  Sum/1 -> Coeff/1
  Constant/1 -> Sum/1
  Matrix Multiply/1 -> Sum/2
  Alpha/1 -> Vector Concatenate/1
  Vector Concatenate/1 -> Matrix Multiply/2
  Constant2/1 -> Matrix Multiply/1
  Beta/1 -> Vector Concatenate/4
  Alpha3/1 -> Vector Concatenate/3
  Alpha2/1 -> Vector Concatenate/2
  Beta2/1 -> Vector Concatenate/5
  Beta3/1 -> Vector Concatenate/6

== system beaver_agent_env/Aerodynamic Model/Aerodynamic Coefficients/Body Rate Damping/Subsystem ==
  V : Inport
  Constant1 : Constant  Value=aircraft.ReferenceSpan
  Constant2 : Constant  Value=aircraft.ReferenceLength
  Divide : Product  Inputs=*/
  Gain1 : Gain  Gain=1/2
  Product : Product  Inputs=*/
  cV : Outport
  b2V : Outport  Port=2
  wires:
  Product/1 -> cV/1
  Constant1/1 -> Gain1/1
  V/1 -> Divide/2, Product/2
  Divide/1 -> b2V/1
  Constant2/1 -> Product/1
  Gain1/1 -> Divide/1
